simulink model "Template_v5_0_0_2026a_Original"  (R2026a)
settings: Solver=ode4  StopTime=tsim  FixedStep=baseRate  RelTol=1e-6  AbsTol=1e-6
undefined symbols (not defined in the file or in its folder): baseRate, dataRate, DiscIntNeverNeededParam, F_thrusters_BLACK, F_thrusters_BLUE, F_thrusters_RED, home_states_BLACK, home_states_BLUE, home_states_RED, IBLACK, IBLUE, init_states_BLACK, init_states_BLUE, init_states_RED, IRED, K_BLACK, K_BLUE, K_RED, labConsoleIP, mBLACK, mBLUE, mRED, Phase0_End, Phase1_End, Phase2_End, Phase3_End, Phase3_SubPhase1_End, Phase3_SubPhase2_End, Phase3_SubPhase3_End, Phase3_SubPhase4_End, Phase4_End, Phase5_End, platformSelection, PWMFreq, serverRate, simMode, tableDamping_BLACK, tableDamping_BLUE, tableDamping_RED, tableSlope, thrust_decay_BLACK, thrust_decay_BLUE, thrust_decay_RED, thruster_dist2CG_BLACK, thruster_dist2CG_BLUE, thruster_dist2CG_RED, xLength, yLength
libraries: simulink x18, dspinverses x3, nvidiaCommlib x1
(part 2 of 7)

== system Template_v5_0_0_2026a_Original/Live Data Streams ==
  note: Each Live Stream block sends what is connected to it to the SPOT Console's Live plot tab, every step, in simulations and experiments. Its name there is the data store's name (or the signal's), unless one is typed into the block. To stream more: copy a Live Stream block and connect a Data Store Read (or any signal) to it.
  Data Store Read : DataStoreRead  DataStoreName=RED_Measured_States  IndexOptions=Index vector (dialog)  Indices=1  OutputSizes=1
  Data Store Read1 : DataStoreRead  DataStoreName=ARM_Measured_States  IndexOptions=Index vector (dialog)  Indices=1  OutputSizes=1
  Data Store Read2 : DataStoreRead  DataStoreName=BLACK_Measured_States  IndexOptions=Index vector (dialog)  Indices=1  OutputSizes=1
  Data Store Read3 : DataStoreRead  DataStoreName=BLUE_Measured_States  IndexOptions=Index vector (dialog)  Indices=1  OutputSizes=1
  Live Stream 1 : Subsystem  mask(Live Stream){streamName=}
      mask prompts: streamName "Name in the live plot (empty: the name of what is connected)"
      mask help: Sends its input to the SPOT Console's Live plot, every step, in simulations and experiments. Its name there is the name of what is connected (e.g. a Data Store Read's data store), unless you type one here. See help spot.hardware.liveStream.
      mask init:
      | streamLabel = uint8(spot.hardware.streamName(gcb, streamName));
      mask Display: disp(['Live: ' char(streamLabel)])
  Live Stream 2 : Subsystem  mask(Live Stream){streamName=}
      mask prompts: streamName "Name in the live plot (empty: the name of what is connected)"
      mask help: Sends its input to the SPOT Console's Live plot, every step, in simulations and experiments. Its name there is the name of what is connected (e.g. a Data Store Read's data store), unless you type one here. See help spot.hardware.liveStream.
      mask init:
      | streamLabel = uint8(spot.hardware.streamName(gcb, streamName));
      mask Display: disp(['Live: ' char(streamLabel)])
  Live Stream 3 : Subsystem  mask(Live Stream){streamName=}
      mask prompts: streamName "Name in the live plot (empty: the name of what is connected)"
      mask help: Sends its input to the SPOT Console's Live plot, every step, in simulations and experiments. Its name there is the name of what is connected (e.g. a Data Store Read's data store), unless you type one here. See help spot.hardware.liveStream.
      mask init:
      | streamLabel = uint8(spot.hardware.streamName(gcb, streamName));
      mask Display: disp(['Live: ' char(streamLabel)])
  Live Stream 4 : Subsystem  mask(Live Stream){streamName=ARM_Measured_States}
      mask prompts: streamName "Name in the live plot (empty: the name of what is connected)"
      mask help: Sends its input to the SPOT Console's Live plot, every step, in simulations and experiments. Its name there is the name of what is connected (e.g. a Data Store Read's data store), unless you type one here. See help spot.hardware.liveStream.
      mask init:
      | streamLabel = uint8(spot.hardware.streamName(gcb, streamName));
      mask Display: disp(['Live: ' char(streamLabel)])
  wires:
  Data Store Read2/1 -> Live Stream 2/1(u)
  Data Store Read/1 -> Live Stream 1/1(u)
  Data Store Read3/1 -> Live Stream 3/1(u)
  Data Store Read1/1 -> Live Stream 4/1(u)

== system Template_v5_0_0_2026a_Original/PhaseSpace Camera Code ==
  note: In this subsection, the "if" statement is used to determine if this is a simulation or not. If it is not a simulation, then code is run to receive PhaseSpace camera data via UDP. The PhaseSpace code is currently a standalone executable that should not need to be modified by most users. The code sends all data for all platforms to each platform near simultaneously. If this is a simulation, then no data is required, but a continuous clock is created.
  Data Store Read2 : DataStoreRead  DataStoreName=isSim  IndexOptions=Index vector (dialog)  Indices=1  OutputSizes=1
  "If performing an experiment, grab the PhaseSpace data. Otherwise, use a clock to set time in SIM." : If  IfExpression=u1 == 0  ElseIfExpressions=u1 == 1  ShowElse=off
  Initialize Universal Time (Simulation) : Subsystem  TreatAsAtomicUnit=on
  Use Hardware to Obtain States : Subsystem  TreatAsAtomicUnit=on
  wires:
  Data Store Read2/1 -> "If performing an experiment, grab the PhaseSpace data. Otherwise, use a clock to set time in SIM."/1
  "If performing an experiment, grab the PhaseSpace data. Otherwise, use a clock to set time in SIM."/2 -> Initialize Universal Time (Simulation)/Action
  "If performing an experiment, grab the PhaseSpace data. Otherwise, use a clock to set time in SIM."/1 -> Use Hardware to Obtain States/Action

== system Template_v5_0_0_2026a_Original/Platform Identification ==
  Data Store Read1 : DataStoreRead  DataStoreName=isSim  IndexOptions=Index vector (dialog)  Indices=1  OutputSizes=1
  "If 'simMode' set to '1', then this is a simulation and the dynamics will be simulated. Otherwise, this is an experiment, and the simulation will not be run." : If  IfExpression=u1 == 0  ShowElse=off
  Subsystem : Subsystem
  wires:
  "If 'simMode' set to '1', then this is a simulation and the dynamics will be simulated. Otherwise, this is an experiment, and the simulation will not be run."/1 -> Subsystem/Action
  Data Store Read1/1 -> "If 'simMode' set to '1', then this is a simulation and the dynamics will be simulated. Otherwise, this is an experiment, and the simulation will not be run."/1

== system Template_v5_0_0_2026a_Original/Receive Data from Orin ==
  Data Store Read1 : DataStoreRead  DataStoreName=isSim  IndexOptions=Index vector (dialog)  Indices=1  OutputSizes=1
  "If 'simMode' set to '1', then this is a simulation and the dynamics will be simulated. Otherwise, this is an experiment, and the simulation will not be run." : If  IfExpression=u1 == 0  ShowElse=off
  Subsystem : Subsystem
  wires:
  "If 'simMode' set to '1', then this is a simulation and the dynamics will be simulated. Otherwise, this is an experiment, and the simulation will not be run."/1 -> Subsystem/Action
  Data Store Read1/1 -> "If 'simMode' set to '1', then this is a simulation and the dynamics will be simulated. Otherwise, this is an experiment, and the simulation will not be run."/1

== system Template_v5_0_0_2026a_Original/Robotic Arm Code ==
  note: This if statement checks if a simulation is being performed. If not, it also checks that this code is being run on the RED platform. If it is, then the arm encoders are used to collect the joint angles. NOTE, the encoder data is collected very slowly, about 0.5 Hz. When the diagram is running faster then this collection rate, previous values of the encoder are held constant.
  PWM : Inport
  Change ARM Behavior : Subsystem  TreatAsAtomicUnit=on
  Data Store Read1 : DataStoreRead  DataStoreName=WhoAmI  IndexOptions=Index vector (dialog)  Indices=1  OutputSizes=1
  Data Store Read2 : DataStoreRead  DataStoreName=isSim  IndexOptions=Index vector (dialog)  Indices=1  OutputSizes=1
  "This IF block determines whether or not to run the RED sim/exp " : If  NumInputs=2  IfExpression=u1 == 1 & u2 == 0  ShowElse=off
  wires:
  Data Store Read2/1 -> "This IF block determines whether or not to run the RED sim/exp "/2
  "This IF block determines whether or not to run the RED sim/exp "/1 -> Change ARM Behavior/Action
  Data Store Read1/1 -> "This IF block determines whether or not to run the RED sim/exp "/1
  PWM/1 -> Change ARM Behavior/1(PWM)

== system Template_v5_0_0_2026a_Original/Send Data to Orin ==
  Data Store Read1 : DataStoreRead  DataStoreName=isSim  IndexOptions=Index vector (dialog)  Indices=1  OutputSizes=1
  "If 'simMode' set to '1', then this is a simulation and the dynamics will be simulated. Otherwise, this is an experiment, and the simulation will not be run." : If  IfExpression=u1 == 0  ShowElse=off
  Subsystem : Subsystem
  wires:
  "If 'simMode' set to '1', then this is a simulation and the dynamics will be simulated. Otherwise, this is an experiment, and the simulation will not be run."/1 -> Subsystem/Action
  Data Store Read1/1 -> "If 'simMode' set to '1', then this is a simulation and the dynamics will be simulated. Otherwise, this is an experiment, and the simulation will not be run."/1

== system Template_v5_0_0_2026a_Original/Simulate Plant Dynamics ==
  Action Port : ActionPort  ActionPortLabel=if(u1 == 1)
  BLACK Dynamics : Subsystem
  BLUE Dynamics : Subsystem
  RED and ARM Dynamics : Subsystem

== system Template_v5_0_0_2026a_Original/Simulation Status ==
  Constant : Constant  Value=simMode  SampleTime=-1
  Data Store Write : DataStoreWrite  DataStoreName=isSim  IndexOptions=Index vector (dialog)  Indices=1  OutputSizes=1
  wires:
  Constant/1 -> Data Store Write/1

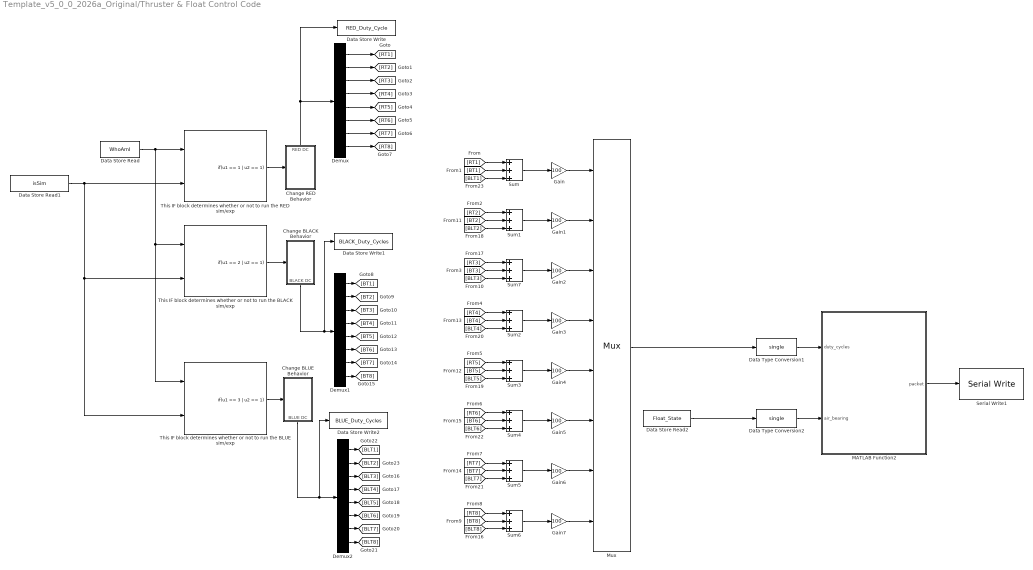
== system Template_v5_0_0_2026a_Original/Thruster & Float Control Code ==
  Change BLACK Behavior : Subsystem  TreatAsAtomicUnit=on
  Change BLUE Behavior : Subsystem  TreatAsAtomicUnit=on
  Change RED Behavior : Subsystem  TreatAsAtomicUnit=on
  Data Store Read : DataStoreRead  DataStoreName=WhoAmI  IndexOptions=Index vector (dialog)  Indices=1  OutputSizes=1
  Data Store Read1 : DataStoreRead  DataStoreName=isSim  IndexOptions=Index vector (dialog)  Indices=1  OutputSizes=1
  Data Store Read2 : DataStoreRead  DataStoreName=Float_State  IndexOptions=Index vector (dialog)  Indices=1  OutputSizes=1
  Data Store Write : DataStoreWrite  DataStoreName=RED_Duty_Cycle  IndexOptions=Index vector (dialog)  Indices=1  OutputSizes=1
  Data Store Write1 : DataStoreWrite  DataStoreName=BLACK_Duty_Cycles  IndexOptions=Index vector (dialog)  Indices=1  OutputSizes=1
  Data Store Write2 : DataStoreWrite  DataStoreName=BLUE_Duty_Cycles  IndexOptions=Index vector (dialog)  Indices=1  OutputSizes=1
  Data Type Conversion1 : DataTypeConversion  OutDataTypeStr=single  SaturateOnIntegerOverflow=off  RndMeth=Floor
  Data Type Conversion2 : DataTypeConversion  OutDataTypeStr=single  SaturateOnIntegerOverflow=off  RndMeth=Floor
  Demux : Demux  Outputs=8
  Demux1 : Demux  Outputs=8
  Demux2 : Demux  Outputs=8
  Gain{,1..7} (8 alike) : Gain  Gain=100
  MATLAB Function2 : MATLAB Function  TreatAsAtomicUnit=on
  Mux : Mux  Inputs=8
  Serial Write1 : nvidiaCommlib/Serial Write  SCIModule=/dev/ttyACM0  Baudrate_=115200  Parity=None  StopBits_=1
  Sum{,1..7} (8 alike) : Sum  Inputs=+++
  This IF block determines whether or not to run the BLACK sim/exp : If  NumInputs=2  IfExpression=u1 == 2 | u2 == 1  ShowElse=off
  This IF block determines whether or not to run the BLUE sim/exp : If  NumInputs=2  IfExpression=u1 == 3 | u2 == 1  ShowElse=off
  "This IF block determines whether or not to run the RED sim/exp " : If  NumInputs=2  IfExpression=u1 == 1 | u2 == 1  ShowElse=off
  wires:
  Data Store Read1/1 -> This IF block determines whether or not to run the BLACK sim/exp/2, This IF block determines whether or not to run the BLUE sim/exp/2, "This IF block determines whether or not to run the RED sim/exp "/2
  "This IF block determines whether or not to run the RED sim/exp "/1 -> Change RED Behavior/Action
  This IF block determines whether or not to run the BLACK sim/exp/1 -> Change BLACK Behavior/Action
  Change RED Behavior/1(RED DC) -> Demux/1, Data Store Write/1
  Demux/1 -> [RT1]
  Demux/2 -> [RT2]
  Demux/3 -> [RT3]
  Demux/4 -> [RT4]
  Demux/5 -> [RT5]
  Demux/6 -> [RT6]
  Demux/7 -> [RT7]
  Demux/8 -> [RT8]
  Demux1/5 -> [BT5]
  Demux1/4 -> [BT4]
  Demux1/1 -> [BT1]
  Demux1/8 -> [BT8]
  Demux1/2 -> [BT2]
  Demux1/7 -> [BT7]
  Demux1/6 -> [BT6]
  Demux1/3 -> [BT3]
  Change BLACK Behavior/1(BLACK DC) -> Demux1/1, Data Store Write1/1
  Data Store Read/1 -> This IF block determines whether or not to run the BLUE sim/exp/1, This IF block determines whether or not to run the BLACK sim/exp/1, "This IF block determines whether or not to run the RED sim/exp "/1
  This IF block determines whether or not to run the BLUE sim/exp/1 -> Change BLUE Behavior/Action
  Demux2/5 -> [BLT5]
  Demux2/8 -> [BLT8]
  Demux2/7 -> [BLT7]
  Demux2/2 -> [BLT2]
  Change BLUE Behavior/1(BLUE DC) -> Data Store Write2/1, Demux2/1
  Demux2/1 -> [BLT1]
  Demux2/4 -> [BLT4]
  Demux2/3 -> [BLT3]
  Demux2/6 -> [BLT6]
  [BT5] -> Sum3/2
  [RT4] -> Sum2/1
  Sum3/1 -> Gain4/1
  [RT2] -> Sum1/1
  [BLT4] -> Sum2/3
  [BT3] -> Sum7/2
  [RT5] -> Sum3/1
  [BT8] -> Sum6/2
  Sum6/1 -> Gain7/1
  Sum7/1 -> Gain2/1
  [BT4] -> Sum2/2
  [RT7] -> Sum5/1
  [BLT3] -> Sum7/3
  [BLT5] -> Sum3/3
  Sum1/1 -> Gain1/1
  Sum2/1 -> Gain3/1
  [BLT6] -> Sum4/3
  [BT6] -> Sum4/2
  [BT2] -> Sum1/2
  [BLT2] -> Sum1/3
  [RT1] -> Sum/1
  Sum/1 -> Gain/1
  [BT7] -> Sum5/2
  [BLT7] -> Sum5/3
  [RT8] -> Sum6/1
  [RT6] -> Sum4/1
  [BLT8] -> Sum6/3
  [BT1] -> Sum/2
  Sum5/1 -> Gain6/1
  Sum4/1 -> Gain5/1
  [BLT1] -> Sum/3
  [RT3] -> Sum7/1
  MATLAB Function2/1(packet) -> Serial Write1/1
  Data Type Conversion1/1 -> MATLAB Function2/1(duty_cycles)
  Data Type Conversion2/1 -> MATLAB Function2/2(air_bearing)
  Data Store Read2/1 -> Data Type Conversion2/1
  Gain/1 -> Mux/1
  Gain1/1 -> Mux/2
  Gain2/1 -> Mux/3
  Gain3/1 -> Mux/4
  Gain4/1 -> Mux/5
  Gain5/1 -> Mux/6
  Gain6/1 -> Mux/7
  Gain7/1 -> Mux/8
  Mux/1 -> Data Type Conversion1/1

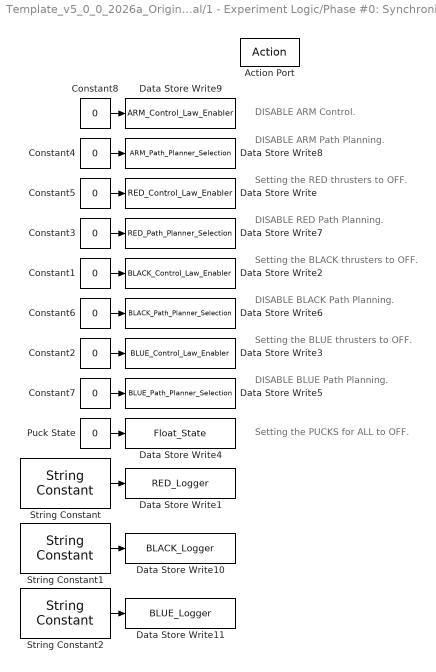
== system Template_v5_0_0_2026a_Original/1 - Experiment Logic/Phase #0: Synchronization ==
  note: Setting the RED thrusters to OFF.
  note: Setting the PUCKS for ALL to OFF.
  note: DISABLE ARM Path Planning.
  note: Setting the BLACK thrusters to OFF.
  note: Setting the BLUE thrusters to OFF.
  note: DISABLE RED Path Planning.
  note: DISABLE BLACK Path Planning.
  note: DISABLE BLUE Path Planning.
  note: DISABLE ARM Control.
  Action Port : ActionPort  ActionPortLabel=if(u1 < u2)
  Constant{1..8} (8 alike) : Constant  Value=0
  Data Store Write : DataStoreWrite  DataStoreName=RED_Control_Law_Enabler  IndexOptions=Index vector (dialog)  Indices=1  OutputSizes=1
  Data Store Write1 : DataStoreWrite  DataStoreName=RED_Logger  IndexOptions=Index vector (dialog)  Indices=1  OutputSizes=1
  Data Store Write10 : DataStoreWrite  DataStoreName=BLACK_Logger  IndexOptions=Index vector (dialog)  Indices=1  OutputSizes=1
  Data Store Write11 : DataStoreWrite  DataStoreName=BLUE_Logger  IndexOptions=Index vector (dialog)  Indices=1  OutputSizes=1
  Data Store Write2 : DataStoreWrite  DataStoreName=BLACK_Control_Law_Enabler  IndexOptions=Index vector (dialog)  Indices=1  OutputSizes=1
  Data Store Write3 : DataStoreWrite  DataStoreName=BLUE_Control_Law_Enabler  IndexOptions=Index vector (dialog)  Indices=1  OutputSizes=1
  Data Store Write4 : DataStoreWrite  DataStoreName=Float_State  IndexOptions=Index vector (dialog)  Indices=1  OutputSizes=1
  Data Store Write5 : DataStoreWrite  DataStoreName=BLUE_Path_Planner_Selection  IndexOptions=Index vector (dialog)  Indices=1  OutputSizes=1
  Data Store Write6 : DataStoreWrite  DataStoreName=BLACK_Path_Planner_Selection  IndexOptions=Index vector (dialog)  Indices=1  OutputSizes=1
  Data Store Write7 : DataStoreWrite  DataStoreName=RED_Path_Planner_Selection  IndexOptions=Index vector (dialog)  Indices=1  OutputSizes=1
  Data Store Write8 : DataStoreWrite  DataStoreName=ARM_Path_Planner_Selection  IndexOptions=Index vector (dialog)  Indices=1  OutputSizes=1
  Data Store Write9 : DataStoreWrite  DataStoreName=ARM_Control_Law_Enabler  IndexOptions=Index vector (dialog)  Indices=1  OutputSizes=1
  Puck State : Constant  Value=0
  String Constant : StringConstant  String="\"Chaser: Running Phase 0\""
  String Constant1 : StringConstant  String="\"Target: Running Phase 0\""
  String Constant2 : StringConstant  String="\"Obstacle: Running Phase 0\""
  wires:
  Constant4/1 -> Data Store Write8/1
  Puck State/1 -> Data Store Write4/1
  Constant5/1 -> Data Store Write/1
  Constant1/1 -> Data Store Write2/1
  Constant2/1 -> Data Store Write3/1
  Constant3/1 -> Data Store Write7/1
  Constant6/1 -> Data Store Write6/1
  Constant7/1 -> Data Store Write5/1
  Constant8/1 -> Data Store Write9/1
  String Constant/1 -> Data Store Write1/1
  String Constant1/1 -> Data Store Write10/1
  String Constant2/1 -> Data Store Write11/1

== system Template_v5_0_0_2026a_Original/1 - Experiment Logic/Phase #1: Start Floating  ==
  note: DISABLE ARM Control.
  note: Setting the BLACK thrusters to OFF.
  note: Setting the PUCKS for ALL to OFF.
  note: DISABLE RED Path Planning.
  note: Setting the RED thrusters to OFF.
  note: Setting the BLUE thrusters to OFF.
  note: DISABLE ARM Path Planning.
  note: DISABLE BLACK Path Planning.
  note: DISABLE BLUE Path Planning.
  Action Port : ActionPort  ActionPortLabel=elseif((u1 < u3 & u1 >= u2))
  Constant{1..8} (8 alike) : Constant  Value=0
  Data Store Write : DataStoreWrite  DataStoreName=RED_Control_Law_Enabler  IndexOptions=Index vector (dialog)  Indices=1  OutputSizes=1
  Data Store Write1 : DataStoreWrite  DataStoreName=RED_Logger  IndexOptions=Index vector (dialog)  Indices=1  OutputSizes=1
  Data Store Write10 : DataStoreWrite  DataStoreName=BLACK_Logger  IndexOptions=Index vector (dialog)  Indices=1  OutputSizes=1
  Data Store Write11 : DataStoreWrite  DataStoreName=BLUE_Logger  IndexOptions=Index vector (dialog)  Indices=1  OutputSizes=1
  Data Store Write2 : DataStoreWrite  DataStoreName=BLACK_Control_Law_Enabler  IndexOptions=Index vector (dialog)  Indices=1  OutputSizes=1
  Data Store Write3 : DataStoreWrite  DataStoreName=BLUE_Control_Law_Enabler  IndexOptions=Index vector (dialog)  Indices=1  OutputSizes=1
  Data Store Write4 : DataStoreWrite  DataStoreName=Float_State  IndexOptions=Index vector (dialog)  Indices=1  OutputSizes=1
  Data Store Write5 : DataStoreWrite  DataStoreName=BLUE_Path_Planner_Selection  IndexOptions=Index vector (dialog)  Indices=1  OutputSizes=1
  Data Store Write6 : DataStoreWrite  DataStoreName=BLACK_Path_Planner_Selection  IndexOptions=Index vector (dialog)  Indices=1  OutputSizes=1
  Data Store Write7 : DataStoreWrite  DataStoreName=RED_Path_Planner_Selection  IndexOptions=Index vector (dialog)  Indices=1  OutputSizes=1
  Data Store Write8 : DataStoreWrite  DataStoreName=ARM_Path_Planner_Selection  IndexOptions=Index vector (dialog)  Indices=1  OutputSizes=1
  Data Store Write9 : DataStoreWrite  DataStoreName=ARM_Control_Law_Enabler  IndexOptions=Index vector (dialog)  Indices=1  OutputSizes=1
  Puck State : Constant
  String Constant : StringConstant  String="\"Chaser: Running Phase 1\""
  String Constant1 : StringConstant  String="\"Target: Running Phase 1\""
  String Constant2 : StringConstant  String="\"Obstacle: Running Phase 1\""
  wires:
  Constant7/1 -> Data Store Write5/1
  Constant2/1 -> Data Store Write3/1
  Constant6/1 -> Data Store Write6/1
  Puck State/1 -> Data Store Write4/1
  Constant1/1 -> Data Store Write2/1
  Constant5/1 -> Data Store Write/1
  Constant3/1 -> Data Store Write7/1
  Constant8/1 -> Data Store Write9/1
  Constant4/1 -> Data Store Write8/1
  String Constant/1 -> Data Store Write1/1
  String Constant1/1 -> Data Store Write10/1
  String Constant2/1 -> Data Store Write11/1

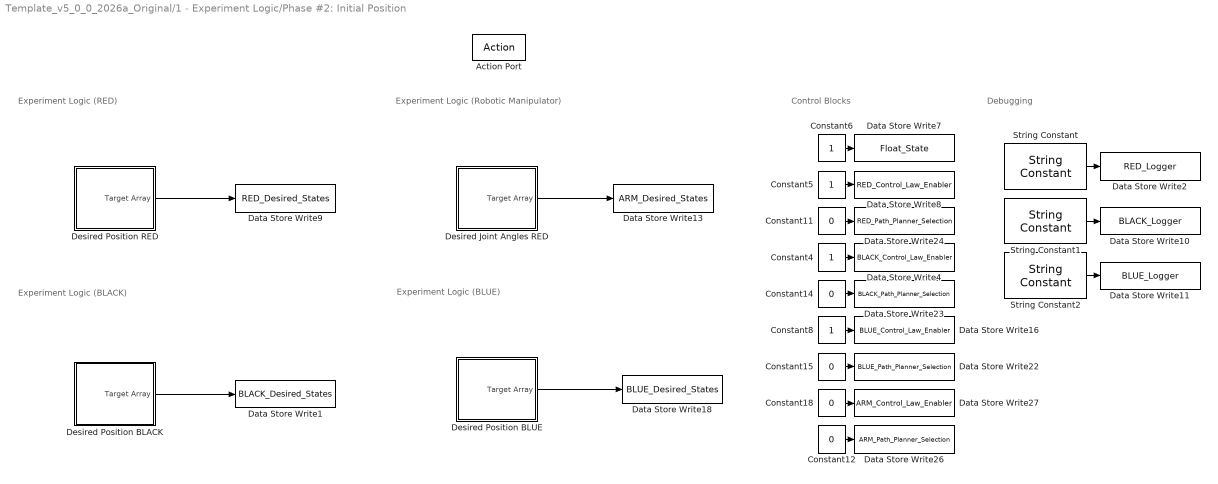
== system Template_v5_0_0_2026a_Original/1 - Experiment Logic/Phase #2: Initial Position ==
  note: Experiment Logic (BLACK)
  note: Control Blocks
  note: Experiment Logic (RED)
  note: Experiment Logic (Robotic Manipulator)
  note: Experiment Logic (BLUE)
  note: Debugging
  Action Port : ActionPort  ActionPortLabel=elseif((u1 < u4 & u1 >= u3))
  Constant{11..12,14..15,18} (5 alike) : Constant  Value=0
  Constant{4..6,8} (4 alike) : Constant
  Data Store Write1 : DataStoreWrite  DataStoreName=BLACK_Desired_States  IndexOptions=Index vector (dialog)  Indices=1  OutputSizes=1
  Data Store Write10 : DataStoreWrite  DataStoreName=BLACK_Logger  IndexOptions=Index vector (dialog)  Indices=1  OutputSizes=1
  Data Store Write11 : DataStoreWrite  DataStoreName=BLUE_Logger  IndexOptions=Index vector (dialog)  Indices=1  OutputSizes=1
  Data Store Write13 : DataStoreWrite  DataStoreName=ARM_Desired_States  IndexOptions=Index vector (dialog)  Indices=1  OutputSizes=1
  Data Store Write16 : DataStoreWrite  DataStoreName=BLUE_Control_Law_Enabler  IndexOptions=Index vector (dialog)  Indices=1  OutputSizes=1
  Data Store Write18 : DataStoreWrite  DataStoreName=BLUE_Desired_States  IndexOptions=Index vector (dialog)  Indices=1  OutputSizes=1
  Data Store Write2 : DataStoreWrite  DataStoreName=RED_Logger  IndexOptions=Index vector (dialog)  Indices=1  OutputSizes=1
  Data Store Write22 : DataStoreWrite  DataStoreName=BLUE_Path_Planner_Selection  IndexOptions=Index vector (dialog)  Indices=1  OutputSizes=1
  Data Store Write23 : DataStoreWrite  DataStoreName=BLACK_Path_Planner_Selection  IndexOptions=Index vector (dialog)  Indices=1  OutputSizes=1
  Data Store Write24 : DataStoreWrite  DataStoreName=RED_Path_Planner_Selection  IndexOptions=Index vector (dialog)  Indices=1  OutputSizes=1
  Data Store Write26 : DataStoreWrite  DataStoreName=ARM_Path_Planner_Selection  IndexOptions=Index vector (dialog)  Indices=1  OutputSizes=1
  Data Store Write27 : DataStoreWrite  DataStoreName=ARM_Control_Law_Enabler  IndexOptions=Index vector (dialog)  Indices=1  OutputSizes=1
  Data Store Write4 : DataStoreWrite  DataStoreName=BLACK_Control_Law_Enabler  IndexOptions=Index vector (dialog)  Indices=1  OutputSizes=1
  Data Store Write7 : DataStoreWrite  DataStoreName=Float_State  IndexOptions=Index vector (dialog)  Indices=1  OutputSizes=1
  Data Store Write8 : DataStoreWrite  DataStoreName=RED_Control_Law_Enabler  IndexOptions=Index vector (dialog)  Indices=1  OutputSizes=1
  Data Store Write9 : DataStoreWrite  DataStoreName=RED_Desired_States  IndexOptions=Index vector (dialog)  Indices=1  OutputSizes=1
  Desired Joint Angles RED : Subsystem
  Desired Position BLACK : Subsystem
  Desired Position BLUE : Subsystem
  Desired Position RED : Subsystem
  String Constant : StringConstant  String="\"Chaser: Running Phase 2\""
  String Constant1 : StringConstant  String="\"Target: Running Phase 2\""
  String Constant2 : StringConstant  String="\"Obstacle: Running Phase 2\""
  wires:
  Constant4/1 -> Data Store Write4/1
  Constant8/1 -> Data Store Write16/1
  Desired Position BLACK/1(Target Array) -> Data Store Write1/1
  Constant5/1 -> Data Store Write8/1
  Desired Position RED/1(Target Array) -> Data Store Write9/1
  Constant6/1 -> Data Store Write7/1
  Desired Position BLUE/1(Target Array) -> Data Store Write18/1
  Constant11/1 -> Data Store Write24/1
  Constant14/1 -> Data Store Write23/1
  Constant15/1 -> Data Store Write22/1
  Desired Joint Angles RED/1(Target Array) -> Data Store Write13/1
  Constant18/1 -> Data Store Write27/1
  Constant12/1 -> Data Store Write26/1
  String Constant1/1 -> Data Store Write10/1
  String Constant2/1 -> Data Store Write11/1
  String Constant/1 -> Data Store Write2/1

== system Template_v5_0_0_2026a_Original/1 - Experiment Logic/Phase #3: Experiment ==
  Action Port : ActionPort  ActionPortLabel=elseif( (u1 < u5 & u1 >= u4))
  Constant1 : Constant  Value=Phase3_SubPhase2_End  SampleTime=-1
  Constant2 : Constant  Value=Phase3_SubPhase3_End  SampleTime=-1
  Constant3 : Constant  Value=Phase3_SubPhase4_End  SampleTime=-1
  Constant4 : Constant  Value=Phase3_SubPhase1_End  SampleTime=-1
  Experiment Sub-Phases : If  NumInputs=5  IfExpression=u1 < u2  ElseIfExpressions=(u1 < u3 & u1 >= u2),(u1 < u4 & u1 >= u3), (u1 < u5 & u1 >= u4)  ShowElse=off
  Sub-Phase #1 : Subsystem  TreatAsAtomicUnit=on
  Sub-Phase #2 : Subsystem  TreatAsAtomicUnit=on
  Sub-Phase #3 : Subsystem  TreatAsAtomicUnit=on
  Sub-Phase #4 : Subsystem  TreatAsAtomicUnit=on
  Universal_Time : DataStoreRead  DataStoreName=Univ_Time  IndexOptions=Index vector (dialog)  Indices=1  OutputSizes=1
  wires:
  Experiment Sub-Phases/3 -> Sub-Phase #3/Action
  Experiment Sub-Phases/4 -> Sub-Phase #4/Action
  Constant3/1 -> Experiment Sub-Phases/5
  Constant2/1 -> Experiment Sub-Phases/4
  Experiment Sub-Phases/1 -> Sub-Phase #1/Action
  Experiment Sub-Phases/2 -> Sub-Phase #2/Action
  Constant1/1 -> Experiment Sub-Phases/3
  Constant4/1 -> Experiment Sub-Phases/2
  Universal_Time/1 -> Experiment Sub-Phases/1

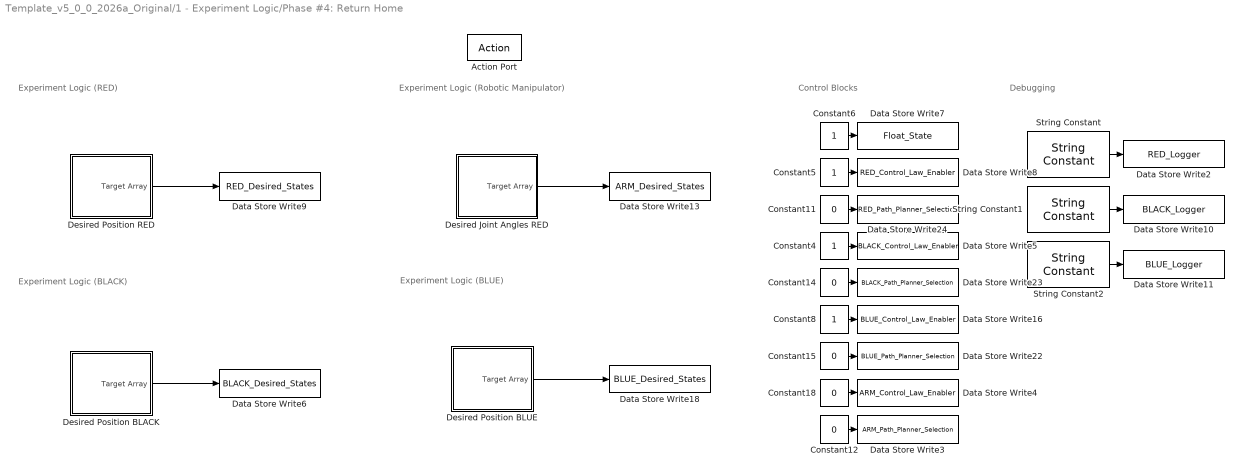
== system Template_v5_0_0_2026a_Original/1 - Experiment Logic/Phase #4: Return Home ==
  note: Experiment Logic (BLACK)
  note: Experiment Logic (Robotic Manipulator)
  note: Experiment Logic (BLUE)
  note: Experiment Logic (RED)
  note: Control Blocks
  note: Debugging
  Action Port : ActionPort  ActionPortLabel=elseif((u1 < u6 & u1 >= u5))
  Constant{11..12,14..15,18} (5 alike) : Constant  Value=0
  Constant{4..6,8} (4 alike) : Constant
  Data Store Write10 : DataStoreWrite  DataStoreName=BLACK_Logger  IndexOptions=Index vector (dialog)  Indices=1  OutputSizes=1
  Data Store Write11 : DataStoreWrite  DataStoreName=BLUE_Logger  IndexOptions=Index vector (dialog)  Indices=1  OutputSizes=1
  Data Store Write13 : DataStoreWrite  DataStoreName=ARM_Desired_States  IndexOptions=Index vector (dialog)  Indices=1  OutputSizes=1
  Data Store Write16 : DataStoreWrite  DataStoreName=BLUE_Control_Law_Enabler  IndexOptions=Index vector (dialog)  Indices=1  OutputSizes=1
  Data Store Write18 : DataStoreWrite  DataStoreName=BLUE_Desired_States  IndexOptions=Index vector (dialog)  Indices=1  OutputSizes=1
  Data Store Write2 : DataStoreWrite  DataStoreName=RED_Logger  IndexOptions=Index vector (dialog)  Indices=1  OutputSizes=1
  Data Store Write22 : DataStoreWrite  DataStoreName=BLUE_Path_Planner_Selection  IndexOptions=Index vector (dialog)  Indices=1  OutputSizes=1
  Data Store Write23 : DataStoreWrite  DataStoreName=BLACK_Path_Planner_Selection  IndexOptions=Index vector (dialog)  Indices=1  OutputSizes=1
  Data Store Write24 : DataStoreWrite  DataStoreName=RED_Path_Planner_Selection  IndexOptions=Index vector (dialog)  Indices=1  OutputSizes=1
  Data Store Write3 : DataStoreWrite  DataStoreName=ARM_Path_Planner_Selection  IndexOptions=Index vector (dialog)  Indices=1  OutputSizes=1
  Data Store Write4 : DataStoreWrite  DataStoreName=ARM_Control_Law_Enabler  IndexOptions=Index vector (dialog)  Indices=1  OutputSizes=1
  Data Store Write5 : DataStoreWrite  DataStoreName=BLACK_Control_Law_Enabler  IndexOptions=Index vector (dialog)  Indices=1  OutputSizes=1
  Data Store Write6 : DataStoreWrite  DataStoreName=BLACK_Desired_States  IndexOptions=Index vector (dialog)  Indices=1  OutputSizes=1
  Data Store Write7 : DataStoreWrite  DataStoreName=Float_State  IndexOptions=Index vector (dialog)  Indices=1  OutputSizes=1
  Data Store Write8 : DataStoreWrite  DataStoreName=RED_Control_Law_Enabler  IndexOptions=Index vector (dialog)  Indices=1  OutputSizes=1
  Data Store Write9 : DataStoreWrite  DataStoreName=RED_Desired_States  IndexOptions=Index vector (dialog)  Indices=1  OutputSizes=1
  Desired Joint Angles RED : Subsystem
  Desired Position BLACK : Subsystem
  Desired Position BLUE : Subsystem
  Desired Position RED : Subsystem
  String Constant : StringConstant  String="\"Chaser: Running Phase 4\""
  String Constant1 : StringConstant  String="\"Target: Running Phase 4\""
  String Constant2 : StringConstant  String="\"Obstacle: Running Phase 4\""
  wires:
  Desired Position RED/1(Target Array) -> Data Store Write9/1
  Desired Position BLACK/1(Target Array) -> Data Store Write6/1
  Desired Position BLUE/1(Target Array) -> Data Store Write18/1
  Constant12/1 -> Data Store Write3/1
  Constant18/1 -> Data Store Write4/1
  Constant6/1 -> Data Store Write7/1
  Constant15/1 -> Data Store Write22/1
  Constant14/1 -> Data Store Write23/1
  Constant5/1 -> Data Store Write8/1
  Constant11/1 -> Data Store Write24/1
  Constant8/1 -> Data Store Write16/1
  Constant4/1 -> Data Store Write5/1
  Desired Joint Angles RED/1(Target Array) -> Data Store Write13/1
  String Constant2/1 -> Data Store Write11/1
  String Constant1/1 -> Data Store Write10/1
  String Constant/1 -> Data Store Write2/1

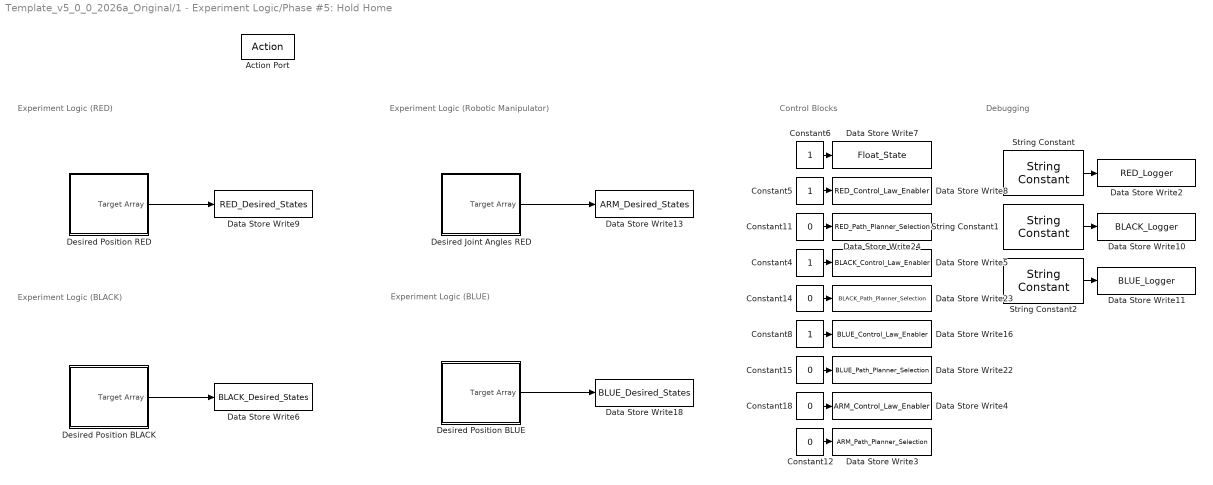
== system Template_v5_0_0_2026a_Original/1 - Experiment Logic/Phase #5: Hold Home ==
  note: Experiment Logic (BLUE)
  note: Experiment Logic (BLACK)
  note: Control Blocks
  note: Experiment Logic (RED)
  note: Experiment Logic (Robotic Manipulator)
  note: Debugging
  Action Port : ActionPort  ActionPortLabel=elseif( (u1 < u7 & u1 >= u6) )
  Constant{11..12,14..15,18} (5 alike) : Constant  Value=0
  Constant{4..6,8} (4 alike) : Constant
  Data Store Write10 : DataStoreWrite  DataStoreName=BLACK_Logger  IndexOptions=Index vector (dialog)  Indices=1  OutputSizes=1
  Data Store Write11 : DataStoreWrite  DataStoreName=BLUE_Logger  IndexOptions=Index vector (dialog)  Indices=1  OutputSizes=1
  Data Store Write13 : DataStoreWrite  DataStoreName=ARM_Desired_States  IndexOptions=Index vector (dialog)  Indices=1  OutputSizes=1
  Data Store Write16 : DataStoreWrite  DataStoreName=BLUE_Control_Law_Enabler  IndexOptions=Index vector (dialog)  Indices=1  OutputSizes=1
  Data Store Write18 : DataStoreWrite  DataStoreName=BLUE_Desired_States  IndexOptions=Index vector (dialog)  Indices=1  OutputSizes=1
  Data Store Write2 : DataStoreWrite  DataStoreName=RED_Logger  IndexOptions=Index vector (dialog)  Indices=1  OutputSizes=1
  Data Store Write22 : DataStoreWrite  DataStoreName=BLUE_Path_Planner_Selection  IndexOptions=Index vector (dialog)  Indices=1  OutputSizes=1
  Data Store Write23 : DataStoreWrite  DataStoreName=BLACK_Path_Planner_Selection  IndexOptions=Index vector (dialog)  Indices=1  OutputSizes=1
  Data Store Write24 : DataStoreWrite  DataStoreName=RED_Path_Planner_Selection  IndexOptions=Index vector (dialog)  Indices=1  OutputSizes=1
  Data Store Write3 : DataStoreWrite  DataStoreName=ARM_Path_Planner_Selection  IndexOptions=Index vector (dialog)  Indices=1  OutputSizes=1
  Data Store Write4 : DataStoreWrite  DataStoreName=ARM_Control_Law_Enabler  IndexOptions=Index vector (dialog)  Indices=1  OutputSizes=1
  Data Store Write5 : DataStoreWrite  DataStoreName=BLACK_Control_Law_Enabler  IndexOptions=Index vector (dialog)  Indices=1  OutputSizes=1
  Data Store Write6 : DataStoreWrite  DataStoreName=BLACK_Desired_States  IndexOptions=Index vector (dialog)  Indices=1  OutputSizes=1
  Data Store Write7 : DataStoreWrite  DataStoreName=Float_State  IndexOptions=Index vector (dialog)  Indices=1  OutputSizes=1
  Data Store Write8 : DataStoreWrite  DataStoreName=RED_Control_Law_Enabler  IndexOptions=Index vector (dialog)  Indices=1  OutputSizes=1
  Data Store Write9 : DataStoreWrite  DataStoreName=RED_Desired_States  IndexOptions=Index vector (dialog)  Indices=1  OutputSizes=1
  Desired Joint Angles RED : Subsystem
  Desired Position BLACK : Subsystem
  Desired Position BLUE : Subsystem
  Desired Position RED : Subsystem
  String Constant : StringConstant  String="\"Chaser: Running Phase 5\""
  String Constant1 : StringConstant  String="\"Target: Running Phase 5\""
  String Constant2 : StringConstant  String="\"Obstacle: Running Phase 5\""
  wires:
  Desired Position RED/1(Target Array) -> Data Store Write9/1
  Desired Position BLACK/1(Target Array) -> Data Store Write6/1
  Desired Position BLUE/1(Target Array) -> Data Store Write18/1
  Constant12/1 -> Data Store Write3/1
  Constant18/1 -> Data Store Write4/1
  Constant6/1 -> Data Store Write7/1
  Constant15/1 -> Data Store Write22/1
  Constant14/1 -> Data Store Write23/1
  Constant5/1 -> Data Store Write8/1
  Constant11/1 -> Data Store Write24/1
  Constant8/1 -> Data Store Write16/1
  Constant4/1 -> Data Store Write5/1
  Desired Joint Angles RED/1(Target Array) -> Data Store Write13/1
  String Constant2/1 -> Data Store Write11/1
  String Constant1/1 -> Data Store Write10/1
  String Constant/1 -> Data Store Write2/1

== system Template_v5_0_0_2026a_Original/1 - Experiment Logic/Phase #6: Clean Shutdown ==
  note: DISABLE ARM Control.
  note: Setting the BLACK thrusters to OFF.
  note: Setting the PUCKS for ALL to OFF.
  note: DISABLE RED Path Planning.
  note: Setting the RED thrusters to OFF.
  note: Setting the BLUE thrusters to OFF.
  note: DISABLE ARM Path Planning.
  note: DISABLE BLACK Path Planning.
  note: DISABLE BLUE Path Planning.
  note: Debugging
  Action Port : ActionPort  ActionPortLabel=elseif((u1 >= u7))
  Constant{1..8} (8 alike) : Constant  Value=0
  Data Store Write : DataStoreWrite  DataStoreName=RED_Control_Law_Enabler  IndexOptions=Index vector (dialog)  Indices=1  OutputSizes=1
  Data Store Write1 : DataStoreWrite  DataStoreName=RED_Logger  IndexOptions=Index vector (dialog)  Indices=1  OutputSizes=1
  Data Store Write10 : DataStoreWrite  DataStoreName=BLACK_Logger  IndexOptions=Index vector (dialog)  Indices=1  OutputSizes=1
  Data Store Write11 : DataStoreWrite  DataStoreName=BLUE_Logger  IndexOptions=Index vector (dialog)  Indices=1  OutputSizes=1
  Data Store Write2 : DataStoreWrite  DataStoreName=BLACK_Control_Law_Enabler  IndexOptions=Index vector (dialog)  Indices=1  OutputSizes=1
  Data Store Write3 : DataStoreWrite  DataStoreName=BLUE_Control_Law_Enabler  IndexOptions=Index vector (dialog)  Indices=1  OutputSizes=1
  Data Store Write4 : DataStoreWrite  DataStoreName=Float_State  IndexOptions=Index vector (dialog)  Indices=1  OutputSizes=1
  Data Store Write5 : DataStoreWrite  DataStoreName=BLUE_Path_Planner_Selection  IndexOptions=Index vector (dialog)  Indices=1  OutputSizes=1
  Data Store Write6 : DataStoreWrite  DataStoreName=BLACK_Path_Planner_Selection  IndexOptions=Index vector (dialog)  Indices=1  OutputSizes=1
  Data Store Write7 : DataStoreWrite  DataStoreName=RED_Path_Planner_Selection  IndexOptions=Index vector (dialog)  Indices=1  OutputSizes=1
  Data Store Write8 : DataStoreWrite  DataStoreName=ARM_Path_Planner_Selection  IndexOptions=Index vector (dialog)  Indices=1  OutputSizes=1
  Data Store Write9 : DataStoreWrite  DataStoreName=ARM_Control_Law_Enabler  IndexOptions=Index vector (dialog)  Indices=1  OutputSizes=1
  Puck State : Constant  Value=0
  String Constant : StringConstant  String="\"Chaser: End of Experiment Reached\""
  String Constant1 : StringConstant  String="\"Target: End of Experiment Reached\""
  String Constant2 : StringConstant  String="\"Obstacle: End of Experiment Reached\""
  wires:
  Constant7/1 -> Data Store Write5/1
  Constant2/1 -> Data Store Write3/1
  Constant6/1 -> Data Store Write6/1
  Puck State/1 -> Data Store Write4/1
  Constant1/1 -> Data Store Write2/1
  Constant5/1 -> Data Store Write/1
  Constant3/1 -> Data Store Write7/1
  Constant8/1 -> Data Store Write9/1
  Constant4/1 -> Data Store Write8/1
  String Constant2/1 -> Data Store Write11/1
  String Constant1/1 -> Data Store Write10/1
  String Constant/1 -> Data Store Write1/1

== system Template_v5_0_0_2026a_Original/3 - Guidance/Custom PPL (ARM) ==
  Action Port : ActionPort  ActionPortLabel=if(u1 == 2)
  Desired Position : Subsystem
  Path : Outport
  wires:
  Desired Position/1(Position Array) -> Path/1

== system Template_v5_0_0_2026a_Original/3 - Guidance/Custom PPL (BLACK) ==
  Action Port : ActionPort  ActionPortLabel=if(u1 == 1 )
  Desired Position : Subsystem
  Path : Outport
  wires:
  Desired Position/1(Position Array) -> Path/1

== system Template_v5_0_0_2026a_Original/3 - Guidance/Custom PPL (BLUE) ==
  Action Port : ActionPort  ActionPortLabel=if(u1 == 2)
  Desired Position : Subsystem
  Path : Outport
  wires:
  Desired Position/1(Position Array) -> Path/1

== system Template_v5_0_0_2026a_Original/3 - Guidance/Custom PPL (RED) ==
  Action Port : ActionPort  ActionPortLabel=if(u1 == 1 )
  Desired Position : Subsystem
  Path : Outport
  wires:
  Desired Position/1(Position Array) -> Path/1

== system Template_v5_0_0_2026a_Original/3 - Guidance/Disable PPL (ARM) ==
  Action Port : ActionPort  ActionPortLabel=else
  Desired Position : Subsystem
  Path : Outport
  wires:
  Desired Position/1(Position Array) -> Path/1

== system Template_v5_0_0_2026a_Original/3 - Guidance/Disable PPL (BLACK) ==
  Action Port : ActionPort  ActionPortLabel=else
  Desired Position : Subsystem
  Path : Outport
  wires:
  Desired Position/1(Position Array) -> Path/1

== system Template_v5_0_0_2026a_Original/3 - Guidance/Disable PPL (BLUE) ==
  Action Port : ActionPort  ActionPortLabel=else
  Desired Position : Subsystem
  Path : Outport
  wires:
  Desired Position/1(Position Array) -> Path/1

== system Template_v5_0_0_2026a_Original/3 - Guidance/Disable PPL (RED) ==
  Action Port : ActionPort  ActionPortLabel=else
  Desired Position : Subsystem
  Path : Outport
  wires:
  Desired Position/1(Position Array) -> Path/1

== system Template_v5_0_0_2026a_Original/4 - Control/Custom Control #1 (BLACK) ==
  Action Port : ActionPort  ActionPortLabel=elseif(u1 == 2)
  Mux1 : Mux  Inputs=3
  Zero1 : Constant  Value=0  OutDataTypeStr=Inherit: Inherit via back propagation
  Out2 : Outport
  wires:
  Zero1/1 -> Mux1/3, Mux1/1, Mux1/2
  Mux1/1 -> Out2/1

== system Template_v5_0_0_2026a_Original/4 - Control/Custom Control #1 (BLUE) ==
  Action Port : ActionPort  ActionPortLabel=elseif(u1 == 2)
  Mux : Mux  Inputs=3
  Zero : Constant  Value=0  OutDataTypeStr=Inherit: Inherit via back propagation
  Out1 : Outport
  wires:
  Mux/1 -> Out1/1
  Zero/1 -> Mux/3, Mux/1, Mux/2

== system Template_v5_0_0_2026a_Original/4 - Control/Custom Control #1 (RED) ==
  Action Port : ActionPort  ActionPortLabel=elseif(u1 == 2)
  Mux : Mux  Inputs=3
  Zero : Constant  Value=0  OutDataTypeStr=Inherit: Inherit via back propagation
  u : Outport
  wires:
  Zero/1 -> Mux/3, Mux/1, Mux/2
  Mux/1 -> u/1

== system Template_v5_0_0_2026a_Original/4 - Control/Custom Control #2 (RED) ==
  Action Port : ActionPort  ActionPortLabel=elseif( u1 == 3)
  Mux : Mux  Inputs=3
  Zero : Constant  Value=0  OutDataTypeStr=Inherit: Inherit via back propagation
  u : Outport
  wires:
  Zero/1 -> Mux/3, Mux/1, Mux/2
  Mux/1 -> u/1

== system Template_v5_0_0_2026a_Original/4 - Control/Custom Control (ARM) ==
  note: PWM control (an example): the path's three values go straight to the servos as joint PWM [885 = 100 % of the supply] (ARM_Controls). At rest PWM acts as a torque (about 0.0068 N m per unit for an MX-64 at 12 V); turning, the motor's back-EMF brakes the joint. Put your own control law here: read ARM_Measured_States (angles, rates) and ARM_Measured_PWM, output three PWM values.
  Action Port : ActionPort  ActionPortLabel=elseif(u1 == 2)
  Calculate PWM : MATLAB Function  TreatAsAtomicUnit=on
  Constant7 : Constant  Value=2
  Data Store Write12 : DataStoreWrite  DataStoreName=ARM_Control_Mode  IndexOptions=Index vector (dialog)  Indices=1  OutputSizes=1
  Goal Speeds (ARM_Path) [rad per s] : DataStoreRead  DataStoreName=ARM_Path  IndexOptions=Index vector (dialog)  Indices=1  OutputSizes=1
  u : Outport
  wires:
  Goal Speeds (ARM_Path) [rad per s]/1 -> Calculate PWM/1(u)
  Calculate PWM/1(y) -> u/1
  Constant7/1 -> Data Store Write12/1

== system Template_v5_0_0_2026a_Original/4 - Control/Default LQR Control (BLACK) ==
  Action Port : ActionPort  ActionPortLabel=if(u1 == 1 )
  Calculate Error : Subsystem
  Constant2 : Constant  Value=-K_BLACK
  Data Store Read1 : DataStoreRead  DataStoreName=BLACK_Path  IndexOptions=Index vector (dialog)  Indices=1  OutputSizes=1
  Data Store Read13 : DataStoreRead  DataStoreName=BLACK_Measured_States  IndexOptions=Index vector (dialog)  Indices=1  OutputSizes=1
  Demux : Demux  Outputs=[1,1,1,1,1,1,3]
  Demux1 : Demux  Outputs=3
  Discrete Derivative : simulink/Discrete/Discrete Derivative  gainval=1.0  ICPrevScaledInput=0.0  OutMin=[]  OutMax=[]  OutDataType=fixdt(1, 16)  OutScaling=2^-10  DoSatur=off
  Discrete Derivative1 : simulink/Discrete/Discrete Derivative  gainval=1.0  ICPrevScaledInput=0.0  OutMin=[]  OutMax=[]  OutDataType=fixdt(1, 16)  OutScaling=2^-10  DoSatur=off
  Discrete Derivative2 : simulink/Discrete/Discrete Derivative  gainval=1.0  ICPrevScaledInput=0.0  OutMin=[]  OutMax=[]  OutDataType=fixdt(1, 16)  OutScaling=2^-10  DoSatur=off
  Matrix Multiply : Product  Multiplication=Matrix(*)
  Mux1 : Mux  Inputs=3
  Mux2 : Mux  Inputs=2
  Mux3 : Mux  Inputs=3
  Reshape1 : Reshape  OutputDimensionality=Column vector (2-D)
  Reshape3 : Reshape  OutputDimensionality=Column vector (2-D)
  Reshape4 : Reshape  OutputDimensionality=Column vector (2-D)
  Subtract{4..8} (5 alike) : Sum  Inputs=-+
  Terminator : Terminator
  u : Outport
  wires:
  Mux2/1 -> Matrix Multiply/2
  Mux1/1 -> Reshape1/1
  Data Store Read13/1 -> Demux/1
  Discrete Derivative2/1 -> Subtract8/1
  Reshape3/1 -> Mux2/2
  Discrete Derivative/1 -> Subtract7/1
  Subtract7/1 -> Mux3/1
  Demux/5 -> Subtract6/2
  Demux1/1 -> Discrete Derivative/1, Subtract5/1
  Demux/2 -> Subtract4/2
  Demux1/3 -> Calculate Error/1(Desired Attitude), Discrete Derivative2/1
  Subtract5/1 -> Mux1/1
  Data Store Read1/1 -> Demux1/1
  Demux/1 -> Subtract5/2
  Mux3/1 -> Reshape3/1
  Demux/6 -> Subtract8/2
  Discrete Derivative1/1 -> Subtract6/1
  Subtract4/1 -> Mux1/2
  Subtract8/1 -> Mux3/3
  Demux/3 -> Calculate Error/2(Measured Attitude)
  Matrix Multiply/1 -> Reshape4/1
  Demux/4 -> Subtract7/2
  Demux1/2 -> Discrete Derivative1/1, Subtract4/1
  Constant2/1 -> Matrix Multiply/1
  Reshape4/1 -> u/1
  Reshape1/1 -> Mux2/1
  Subtract6/1 -> Mux3/2
  Calculate Error/1(Attitude Error) -> Mux1/3
  Demux/7 -> Terminator/1

== system Template_v5_0_0_2026a_Original/4 - Control/Default LQR Control (BLUE) ==
  Action Port : ActionPort  ActionPortLabel=if(u1 == 1 )
  Calculate Error : Subsystem
  Constant2 : Constant  Value=-K_BLUE
  Data Store Read1 : DataStoreRead  DataStoreName=BLUE_Path  IndexOptions=Index vector (dialog)  Indices=1  OutputSizes=1
  Data Store Read2 : DataStoreRead  DataStoreName=BLUE_Measured_States  IndexOptions=Index vector (dialog)  Indices=1  OutputSizes=1
  Demux : Demux  Outputs=[1,1,1,1,1,1,3]
  Demux1 : Demux  Outputs=3
  Discrete Derivative : simulink/Discrete/Discrete Derivative  gainval=1.0  ICPrevScaledInput=0.0  OutMin=[]  OutMax=[]  OutDataType=fixdt(1, 16)  OutScaling=2^-10  DoSatur=off
  Discrete Derivative1 : simulink/Discrete/Discrete Derivative  gainval=1.0  ICPrevScaledInput=0.0  OutMin=[]  OutMax=[]  OutDataType=fixdt(1, 16)  OutScaling=2^-10  DoSatur=off
  Discrete Derivative2 : simulink/Discrete/Discrete Derivative  gainval=1.0  ICPrevScaledInput=0.0  OutMin=[]  OutMax=[]  OutDataType=fixdt(1, 16)  OutScaling=2^-10  DoSatur=off
  Matrix Multiply : Product  Multiplication=Matrix(*)
  Mux : Mux  Inputs=3
  Mux1 : Mux  Inputs=2
  Mux2 : Mux  Inputs=3
  Reshape1 : Reshape  OutputDimensionality=Column vector (2-D)
  Reshape2 : Reshape  OutputDimensionality=Column vector (2-D)
  Reshape4 : Reshape  OutputDimensionality=Column vector (2-D)
  Subtract{4..8} (5 alike) : Sum  Inputs=-+
  Terminator : Terminator
  u : Outport
  wires:
  Demux1/3 -> Calculate Error/1(Desired Attitude), Discrete Derivative2/1
  Discrete Derivative/1 -> Subtract7/1
  Reshape4/1 -> u/1
  Demux/7 -> Terminator/1
  Demux/5 -> Subtract6/2
  Subtract6/1 -> Mux2/2
  Demux/4 -> Subtract7/2
  Subtract4/1 -> Mux/2
  Mux2/1 -> Reshape2/1
  Demux/6 -> Subtract8/2
  Reshape2/1 -> Mux1/2
  Demux/2 -> Subtract4/2
  Calculate Error/1(Attitude Error) -> Mux/3
  Mux/1 -> Reshape1/1
  Subtract8/1 -> Mux2/3
  Discrete Derivative2/1 -> Subtract8/1
  Demux/3 -> Calculate Error/2(Measured Attitude)
  Mux1/1 -> Matrix Multiply/2
  Data Store Read1/1 -> Demux1/1
  Demux1/1 -> Discrete Derivative/1, Subtract5/1
  Data Store Read2/1 -> Demux/1
  Demux/1 -> Subtract5/2
  Reshape1/1 -> Mux1/1
  Subtract5/1 -> Mux/1
  Demux1/2 -> Discrete Derivative1/1, Subtract4/1
  Discrete Derivative1/1 -> Subtract6/1
  Subtract7/1 -> Mux2/1
  Matrix Multiply/1 -> Reshape4/1
  Constant2/1 -> Matrix Multiply/1

== system Template_v5_0_0_2026a_Original/4 - Control/Default LQR Control (RED) ==
  Action Port : ActionPort  ActionPortLabel=if(u1 == 1 )
  Calculate Error : Subsystem
  Constant2 : Constant  Value=-K_RED
  Data Store Read1 : DataStoreRead  DataStoreName=RED_Path  IndexOptions=Index vector (dialog)  Indices=1  OutputSizes=1
  Data Store Read13 : DataStoreRead  DataStoreName=RED_Measured_States  IndexOptions=Index vector (dialog)  Indices=1  OutputSizes=1
  Demux : Demux  Outputs=[1,1,1,1,1,1,3]
  Demux1 : Demux  Outputs=3
  Discrete Derivative : simulink/Discrete/Discrete Derivative  gainval=1.0  ICPrevScaledInput=0.0  OutMin=[]  OutMax=[]  OutDataType=fixdt(1, 16)  OutScaling=2^-10  DoSatur=off
  Discrete Derivative1 : simulink/Discrete/Discrete Derivative  gainval=1.0  ICPrevScaledInput=0.0  OutMin=[]  OutMax=[]  OutDataType=fixdt(1, 16)  OutScaling=2^-10  DoSatur=off
  Discrete Derivative2 : simulink/Discrete/Discrete Derivative  gainval=1.0  ICPrevScaledInput=0.0  OutMin=[]  OutMax=[]  OutDataType=fixdt(1, 16)  OutScaling=2^-10  DoSatur=off
  Matrix Multiply : Product  Multiplication=Matrix(*)
  Mux1 : Mux  Inputs=3
  Mux2 : Mux  Inputs=2
  Mux3 : Mux  Inputs=3
  Reshape2 : Reshape  OutputDimensionality=Column vector (2-D)
  Reshape3 : Reshape  OutputDimensionality=Column vector (2-D)
  Reshape4 : Reshape  OutputDimensionality=Column vector (2-D)
  Subtract{4..8} (5 alike) : Sum  Inputs=-+
  Terminator : Terminator
  u : Outport
  wires:
  Subtract7/1 -> Mux3/1
  Constant2/1 -> Matrix Multiply/1
  Subtract5/1 -> Mux1/1
  Calculate Error/1(Attitude Error) -> Mux1/3
  Reshape3/1 -> Mux2/2
  Demux/3 -> Calculate Error/2(Measured Attitude)
  Data Store Read1/1 -> Demux1/1
  Mux2/1 -> Matrix Multiply/2
  Reshape2/1 -> Mux2/1
  Subtract4/1 -> Mux1/2
  Data Store Read13/1 -> Demux/1
  Matrix Multiply/1 -> Reshape4/1
  Subtract6/1 -> Mux3/2
  Demux/7 -> Terminator/1
  Mux3/1 -> Reshape3/1
  Subtract8/1 -> Mux3/3
  Demux/2 -> Subtract4/2
  Demux1/2 -> Discrete Derivative1/1, Subtract4/1
  Mux1/1 -> Reshape2/1
  Discrete Derivative2/1 -> Subtract8/1
  Demux1/3 -> Calculate Error/1(Desired Attitude), Discrete Derivative2/1
  Discrete Derivative/1 -> Subtract7/1
  Demux/6 -> Subtract8/2
  Demux1/1 -> Discrete Derivative/1, Subtract5/1
  Demux/4 -> Subtract7/2
  Demux/5 -> Subtract6/2
  Reshape4/1 -> u/1
  Demux/1 -> Subtract5/2
  Discrete Derivative1/1 -> Subtract6/1

== system Template_v5_0_0_2026a_Original/4 - Control/Default Position Control (ARM) ==
  note: Default arm control: the path's joint angles (ARM_Path) are goal positions (ARM_Control_Mode = 1). spot.control.ArmPositionControl runs the servos' own position law (profile, PID) here, in the diagram, and gives each joint's PWM (ARM_Controls), in simulation and on the hardware.
  Action Port : ActionPort  InitializeStates=reset  ActionPortLabel=if(u1 == 1 )
  Constant7 : Constant
  Data Store Read1 : DataStoreRead  DataStoreName=ARM_Measured_States  IndexOptions=Index vector (dialog)  Indices=1  OutputSizes=1
  Data Store Read2 : DataStoreRead  DataStoreName=ARM_Path  IndexOptions=Index vector (dialog)  Indices=1  OutputSizes=1
  Data Store Write12 : DataStoreWrite  DataStoreName=ARM_Control_Mode  IndexOptions=Index vector (dialog)  Indices=1  OutputSizes=1
  Dynamixel Position Control : MATLABSystem  System=spot.control.ArmPositionControl  StepTime=baseRate  ServoPeriod=1e-3  PositionP=armControl.position.P  PositionI=armControl.position.I  PositionD=armControl.position.D  Feedforward1=0  Feedforward2=0  ProfileVelocity=armControl.position.profileVelocity  ProfileAcceleration=armControl.position.profileAcceleration  MinPosition=1024  MaxPosition=3072  PWMLimit=armControl.position.pwmLimit  SimulateUsing=Code generation
      mask Type: spot.control.ArmPositionControl
  u : Outport
  wires:
  Constant7/1 -> Data Store Write12/1
  Data Store Read2/1 -> Dynamixel Position Control/1
  Data Store Read1/1 -> Dynamixel Position Control/2
  Dynamixel Position Control/1 -> u/1

== system Template_v5_0_0_2026a_Original/4 - Control/Default Velocity Control (ARM) ==
  note: The path's three values are goal joint speeds [rad/s] here (spot.control.ArmVelocityControl: the servo's velocity law, giving each joint's PWM).
  Action Port : ActionPort  InitializeStates=reset  ActionPortLabel=elseif( u1 == 3)
  Constant7 : Constant  Value=3
  Data Store Write12 : DataStoreWrite  DataStoreName=ARM_Control_Mode  IndexOptions=Index vector (dialog)  Indices=1  OutputSizes=1
  Dynamixel Velocity Control : MATLABSystem  System=spot.control.ArmVelocityControl  StepTime=baseRate  ServoPeriod=1e-3  VelocityP=armControl.velocity.P  VelocityI=armControl.velocity.I  ProfileAcceleration=armControl.velocity.profileAcceleration  VelocityLimit=1023  PWMLimit=armControl.velocity.pwmLimit  SimulateUsing=Code generation
      mask Type: spot.control.ArmVelocityControl
  Goal Speeds (ARM_Path) [rad per s] : DataStoreRead  DataStoreName=ARM_Path  IndexOptions=Index vector (dialog)  Indices=1  OutputSizes=1
  Goal Speeds (ARM_Path) [rad per s]1 : DataStoreRead  DataStoreName=ARM_Measured_States  IndexOptions=Index vector (dialog)  Indices=1  OutputSizes=1
  u : Outport
  wires:
  Dynamixel Velocity Control/1 -> u/1
  Goal Speeds (ARM_Path) [rad per s]1/1 -> Dynamixel Velocity Control/2
  Goal Speeds (ARM_Path) [rad per s]/1 -> Dynamixel Velocity Control/1
  Constant7/1 -> Data Store Write12/1
